simulink model "s_c_nbe_m32k"  (R2018a)
settings: Solver=VariableStepDiscrete  StartTime=0.0  StopTime=1000  RelTol=1e-3
undefined symbols (not defined in the file): fft_stages, n_taps, output_bits, pfb_coeff_gen_calc, xengbits
libraries: xbsIndex_r4 x23714, casper_library_misc x17, xps_library x4, casper_library_scopes x4, xbsReplacements_r4 x4
(part 85 of 171)

== system s_c_nbe_m32k/nb_pfb/pfb_fir_generic1/pfb_fir_taps ==
  sync : Inport
  din : Inport  Port=2
  coeffs : Inport  Port=3
  en : Inport  Port=4
  arnold : Terminator
  bram_din : xbsIndex_r4/Concat  num_inputs=2  dbl_ovrd=off  block_type=concat
  bus_adder_tree : Subsystem  mask(bus_adder_tree){n_busses=4, n_bits=[36 36], num_float_vec=1, bin_pts=34, dtypes=1, misc=off, floating_point=off, float_type=single, frac_width=24, exp_width=8, add_latency=7, first_stage_hdl=on, adder_imp=Behavioral}
      mask prompts: n_busses "number of busses"; n_bits "bus component bit widths"; num_float_vec "number floating point vectors in bus"; bin_pts "bus component binary points"; dtypes "bus component data types"; misc "misc support"; floating_point "floating point"; float_type "float type"; frac_width "fraction width"; exp_width "exponent width"; add_latency "adder latency"; first_stage_hdl "implement first stage in of adders in behavioral HDL?"; adder_imp "adder implementation"
      mask help: Add components of multiple identical busses
      mask init:
      | bus_adder_tree_init(gcb, ...
      |     'n_busses', n_busses, ...
      |     'n_bits', n_bits, ...
      |     'bin_pts', bin_pts, ...
      |     'dtypes', dtypes, ...
      |     'add_latency', add_latency, ...
      |     'floating_point', floating_point, ...
      |     'float_type', float_type, ...
      |     'exp_width', exp_width, ...
      |     'frac_width', frac_width, ...   
      |     'num_float_vec', num_float_vec, ...
      |     'first_stage_hdl', first_stage_hdl, ...
      |     'adder_imp', adder_imp, ...
      |     'misc', misc);
      mask Callback floating_point:
      | onoff = get_param(gcb, 'floating_point');
      | if strcmp(onoff,'on')
      |     enable_fixpt = 'off'
      |     set_param_state(gcb, 'float_type', 'on')
      |     set_param_state(gcb, 'num_float_vec', 'on')
      | 
      |     f_type = get_param(gcb, 'float_type')
      |     if strcmp(f_type,'custom')
      |         set_param_state(gcb, 'exp_width', 'on')
      |         set_param_state(gcb, 'frac_width', 'on')
      |     else
      |         set_param_state(gcb, 'exp_width', 'off')
      |         set_param_state(gcb, 'frac_width', 'off')
      |     end
      | 
      | 
      | else
      |     enable_fixpt = 'on'
      |     set_param_state(gcb, 'float_type', 'off')
      |     set_param_state(gcb, 'exp_width', 'off')
      |     set_param_state(gcb, 'frac_width', 'off')
      |     set_param_state(gcb, 'num_float_vec', 'off')
      | end
      | 
      | set_param_state(gcb, 'n_bits', enable_fixpt)
      | set_param_state(gcb, 'bin_pts', enable_fixpt)
      | set_param_state(gcb, 'dtypes', enable_fixpt)
      mask TypeOptions float_type: single | custom
      mask Callback float_type:
      | f_type = get_param(gcb, 'float_type')
      | if strcmp(f_type,'custom')
      |     set_param_state(gcb, 'exp_width', 'on')
      |     set_param_state(gcb, 'frac_width', 'on')
      | else
      |     set_param_state(gcb, 'exp_width', 'off')
      |     set_param_state(gcb, 'frac_width', 'off')
      | end
      mask TypeOptions adder_imp: Behavioral | Fabric | DSP48
  bus_mult : Subsystem  mask(bus_mult){n_bits_a=[18 18 18 18 18 18 18 18], bin_pt_a=17, type_a=1, cmplx_a=off, n_bits_b=[18 18 18 18 18 18 18 18], bin_pt_b=17, type_b=1, cmplx_b=off, misc=off, floating_point=off, float_type=single, input_vec_a=1, input_vec_b=1, frac_width=24, exp_width=8, n_bits_out=n_bits_data+n_bits_coeff, bin_pt_out=n_bits_data-1+bin_pt_coeff, type_out=1, quantization=0, overflow=0, mult_latency=mult_latency, add_latency=0, conv_latency=0, max_fanout=1, fan_latency=0, multiplier_implementation=behavioral HDL, pipeline_cmult_en=off, pipeline_latency=0}
      mask prompts: n_bits_a "a input bit widths"; bin_pt_a "a input binary points"; type_a "a input type (Unsigned=0, Signed=1)"; cmplx_a "a input complex"; n_bits_b "b input bit widths"; bin_pt_b "b input binary points"; type_b "b input type (Unsigned=0, Signed=1)"; cmplx_b "b input complex"; misc "misc support"; floating_point "floating point"; float_type "float type"; input_vec_a "a input vector in bus"; input_vec_b "b input vector in bus"; frac_width "fraction width"; exp_width "exponent width"; n_bits_out "output bit widths"; bin_pt_out "output binary points"; type_out "output type (Unsigned=0, Signed=1)"; quantization "quantization strategy (Truncate=0, Round  (unbiased: +/- Inf)=1)"; overflow "overflow strategy (Wrap=0, Saturate=1, Flag as error=2)"; mult_latency "multiplier latency"; add_latency "adder latency"; conv_latency "convert latency"; max_fanout "limit fanout to ?"; fan_latency "fanout register latency"; multiplier_implementation "multiplier implementation"; pipeline_cmult_en "pipeline complex mult"; pipeline_latency "pipeline latency"
      mask help: Multiply components of two busses
      mask init: same as s_c_nbe_m32k/DDC/bus_mult
      mask Callback floating_point:
      | onoff = get_param(gcb, 'floating_point');
      | if strcmp(onoff,'on')
      |     enable_fixpt = 'off'
      |     set_param_state(gcb, 'float_type', 'on')
      | 
      |     set_param_state(gcb, 'input_vec_a', 'on')
      |     set_param_state(gcb, 'input_vec_b', 'on')
      | 
      |     f_type = get_param(gcb, 'float_type')
      |     if strcmp(f_type,'custom')
      |         set_param_state(gcb, 'exp_width', 'on')
      |         set_param_state(gcb, 'frac_width', 'on')
      |     else
      |         set_param_state(gcb, 'exp_width', 'off')
      |         set_param_state(gcb, 'frac_width', 'off')
      |     end
      | 
      | else
      |     enable_fixpt = 'on'
      |     set_param_state(gcb, 'float_type', 'off')
      |     set_param_state(gcb, 'exp_width', 'off')
      |     set_param_state(gcb, 'frac_width', 'off')
      |     set_param_state(gcb, 'input_vec_a', 'off')
      |     set_param_state(gcb, 'input_vec_b', 'off')
      | end
      | 
      | set_param_state(gcb, 'n_bits_a', enable_fixpt)
      | set_param_state(gcb, 'bin_pt_a', enable_fixpt)
      | set_param_state(gcb, 'type_a', enable_fixpt)
      | set_param_state(gcb, 'n_bits_b', enable_fixpt)
      | set_param_state(gcb, 'bin_pt_b', enable_fixpt)
      | set_param_state(gcb, 'type_b', enable_fixpt)
      | 
      | set_param_state(gcb, 'n_bits_out', enable_fixpt)
      | set_param_state(gcb, 'bin_pt_out', enable_fixpt)
      | set_param_state(gcb, 'type_out', enable_fixpt)
      | set_param_state(gcb, 'quantization', enable_fixpt)
      | set_param_state(gcb, 'overflow', enable_fixpt)
      mask TypeOptions float_type: single | custom
      mask Callback float_type:
      | f_type = get_param(gcb, 'float_type')
      | if strcmp(f_type,'custom')
      |     set_param_state(gcb, 'exp_width', 'on')
      |     set_param_state(gcb, 'frac_width', 'on')
      | else
      |     set_param_state(gcb, 'exp_width', 'off')
      |     set_param_state(gcb, 'frac_width', 'off')
      | end
      mask TypeOptions multiplier_implementation: behavioral HDL | standard core | embedded multiplier core
      mask Callback pipeline_cmult_en:
      | pipeline_en = get_param(gcb, 'pipeline_cmult_en');
      | if strcmp(pipeline_en,'on')
      | 
      |     set_param_state(gcb, 'pipeline_latency', 'on')
      | else
      |     set_param_state(gcb, 'pipeline_latency', 'off')
      | end
  counter : xbsIndex_r4/Counter  cnt_type=Free Running  cnt_to=Inf  operation=Up  start_count=0  cnt_by_val=1  arith_type=Unsigned  n_bits=15  bin_pt=0  load_pin=off  rst=on  en=on  explicit_period=on  period=1  use_behavioral_HDL=off  implementation=Fabric  dbl_ovrd=off  block_type=counter
  daddr : xbsIndex_r4/Delay  rst=off  infoeditControl=Selection of Reset will increase slice count due to use of real FFs and instead of SRLs  en=off  latency=11  reg_retiming=on  dbl_ovrd=off  block_type=delay
  dcoeffs : xbsIndex_r4/Delay  rst=off  infoeditControl=Selection of Reset will increase slice count due to use of real FFs and instead of SRLs  en=off  latency=11  reg_retiming=on  dbl_ovrd=off  block_type=delay
  ddin : xbsIndex_r4/Delay  rst=off  infoeditControl=Selection of Reset will increase slice count due to use of real FFs and instead of SRLs  en=off  latency=11  reg_retiming=off  dbl_ovrd=off  block_type=delay
  den0 : xbsIndex_r4/Delay  rst=off  infoeditControl=Selection of Reset will increase slice count due to use of real FFs and instead of SRLs  en=off  latency=11  reg_retiming=on  dbl_ovrd=off  block_type=delay
  den1 : xbsIndex_r4/Delay  rst=off  infoeditControl=Selection of Reset will increase slice count due to use of real FFs and instead of SRLs  en=off  latency=7  reg_retiming=on  dbl_ovrd=off  block_type=delay
  den2 : xbsIndex_r4/Delay  rst=off  infoeditControl=Selection of Reset will increase slice count due to use of real FFs and instead of SRLs  en=off  latency=14  reg_retiming=on  dbl_ovrd=off  block_type=delay
  dsync0 : xbsIndex_r4/Delay  rst=off  infoeditControl=Selection of Reset will increase slice count due to use of real FFs and instead of SRLs  en=off  latency=11  reg_retiming=on  dbl_ovrd=off  block_type=delay
  dsync1 : xbsIndex_r4/Delay  rst=off  infoeditControl=Selection of Reset will increase slice count due to use of real FFs and instead of SRLs  en=off  latency=7  reg_retiming=on  dbl_ovrd=off  block_type=delay
  dsync2 : xbsIndex_r4/Delay  rst=off  infoeditControl=Selection of Reset will increase slice count due to use of real FFs and instead of SRLs  en=off  latency=14  reg_retiming=on  dbl_ovrd=off  block_type=delay
  mult_din : xbsIndex_r4/Concat  num_inputs=2  dbl_ovrd=off  block_type=concat
  never : xbsIndex_r4/Constant  const=0  gui_display_data_type=Fixed-point  arith_type=Boolean  n_bits=16  bin_pt=14  preci_type=Single  exp_width=8  frac_width=24  explicit_period=on  period=1  equ=P=C  opselect=C  inp2=PCIN>>17  opr=+  inp1=P  carry=CIN  dbl_ovrd=off  block_type=constant
  sync_delay1 : Subsystem  mask(sync_delay_en){DelayLen=(2^(pfb_size-n_inputs))*(n_taps-1)}
      mask prompts: DelayLen "Delay Length:"
      mask help: Delay an infrequent boolean pulse by the specified number of enabled clocks.
      mask init:
      | BitWidth = max(2, ceil(log2(DelayLen+1)));
      | UseCounter = 1;
      | if DelayLen == 0,
      | 	UseCounter = 0;
      | end
      mask Help: eval('xlWeb(''http://casper.berkeley.edu/wiki/Sync_delay_en'')')
      mask Display:
      | fprintf('Z^-%d', DelayLen);
      | port_label('input',2,'en');
  tap_delays : Subsystem  mask(bus_dual_port_ram){n_bits=[18 18 18 18 18 18], bin_pts=[0 0 0 0 0 0], init_vector=repmat(zeros(32768, 1), 1, 6), max_fanout=1, mem_type=Block RAM, bram_optimization=Speed, async_a=off, async_b=off, b_to_a_ratio_bits=0, misc=off, bram_latency=7, fan_latency=4, addra_register=on, addra_implementation=core, dina_register=off, dina_implementation=behavioral, wea_register=off, wea_implementation=behavioral, ena_register=off, ena_implementation=behavioral, addrb_register=on, addrb_implementation=core, dinb_register=on, dinb_implementation=core, web_register=on, web_implementation=core, enb_register=off, enb_implementation=behavioral}
      mask prompts: n_bits "data word bit widths"; bin_pts "data word binary points"; init_vector "initial value vector"; max_fanout "limit fanout to ?"; mem_type "memory type"; bram_optimization "memory optimization"; async_a "a asynchronous"; async_b "b asynchronous"; b_to_a_ratio_bits "b_to_a ratio bits"; misc "misc support"; bram_latency "bram latency"; fan_latency "input register latency"; addra_register "addra input register"; addra_implementation "addra register implementation"; dina_register "dina input register"; dina_implementation "dina register implementation"; wea_register "wea input register"; wea_implementation "wea register implementation"; ena_register "ena input register"; ena_implementation "ena register implementation"; addrb_register "addrb input register"; addrb_implementation "addrb register implementation"; dinb_register "dinb input register"; dinb_implementation "dinb register implementation"; web_register "web input register"; web_implementation "web register implementation"; enb_register "enb input register"; enb_implementation "enb register implementation"
      mask help: RAM for a bus allowing fanout control
      mask init: same as s_c_nbe_m32k/nb_pfb/pfb_fir_generic1/pfb_fir_coeff_gen/rom
      mask TypeOptions mem_type: Distributed memory | Block RAM
      mask TypeOptions bram_optimization: Area | Speed
      mask TypeOptions addra_implementation: core | behavioral
      mask TypeOptions dina_implementation: core | behavioral
      mask TypeOptions wea_implementation: core | behavioral
      mask TypeOptions ena_implementation: core | behavioral
      mask TypeOptions addrb_implementation: core | behavioral
      mask TypeOptions dinb_implementation: core | behavioral
      mask TypeOptions web_implementation: core | behavioral
      mask TypeOptions enb_implementation: core | behavioral
  tap_split : Subsystem  mask(bus_expand){mode=divisions of equal size, outputNum=4, outputWidth=72, outputBinaryPt=0, outputArithmeticType=0, show_format=off, outputToWorkspace=off, variablePrefix=out, outputToModelAsWell=on}
      mask prompts: outputNum "Number of outputs:"; outputWidth "Output width:"; outputBinaryPt "Output binary point position:"; outputArithmeticType "Output arithmetic type (ufix=0, fix=1, bool=2):"; show_format "Print format string?"; outputToWorkspace "Output to workspace?"; variablePrefix "Variable name prefix:"; outputToModelAsWell "Output to model as well?"
      mask help:
      | Expands a 'bus' made using a bus_create or Xilinx
      | concat block.
      | The input will be divided into the specified number
      | of outputs with the specified arithmetic types.
      | Divisions are made from most significant bit.
      mask init: same as s_c_nbe_m32k/bus_expand1
      settings: AttributesFormatString=4 outputs
      mask TypeOptions mode: divisions of equal size | divisions of arbitrary size
      mask Callback mode: bus_expand_callback();
      mask Callback outputWidth: bus_expand_callback();
      mask Callback outputToWorkspace: bus_expand_callback();
  youngest : xbsIndex_r4/Slice  nbits=(2*n_bits_data)*(n_taps-2)*(2^n_inputs)*n_streams  boolean_output=off  mode=Upper Bit Location + Width  bit1=0  base1=MSB of Input  bit0=0  base0=LSB of Input  dbl_ovrd=off  block_type=slice
  sync_out : Outport
  dout : Outport  Port=2
  dvalid : Outport  Port=3
  wires:
  dsync0/1 -> dsync1/1
  dsync1/1 -> dsync2/1
  dsync2/1 -> sync_out/1
  din/1 -> ddin/1
  coeffs/1 -> dcoeffs/1
  en/1 -> sync_delay1/2(en), den0/1, counter/2
  den0/1 -> den1/1, tap_delays/6(web)
  den1/1 -> den2/1
  sync/1 -> sync_delay1/1(In), counter/1
  sync_delay1/1(Out) -> dsync0/1
  ddin/1 -> bram_din/1, mult_din/1
  youngest/1 -> bram_din/2
  counter/1 -> daddr/1, tap_delays/1(addra)
  bram_din/1 -> tap_delays/2(dina), tap_delays/5(dinb)
  never/1 -> tap_delays/3(wea)
  daddr/1 -> tap_delays/4(addrb)
  tap_delays/2(B) -> arnold/1
  tap_delays/1(A) -> mult_din/2, youngest/1
  mult_din/1 -> bus_mult/1(a)
  dcoeffs/1 -> bus_mult/2(b)
  bus_mult/1(a*b) -> tap_split/1(bus_in)
  tap_split/1(msb_out4) -> bus_adder_tree/1(d0)
  tap_split/2(out3) -> bus_adder_tree/2(d1)
  tap_split/3(out2) -> bus_adder_tree/3(d2)
  tap_split/4(lsb_out1) -> bus_adder_tree/4(d3)
  bus_adder_tree/1(out) -> dout/1
  den2/1 -> dvalid/1

== system s_c_nbe_m32k/nb_pfb/pfb_fir_generic2/bus_convert ==
  din : Inport
  bussify : Subsystem  mask(bus_create){inputNum=2}
      mask prompts: inputNum "Number of inputs:"
      mask init:
      | bus_create_init(gcb,...
      |     'inputNum', inputNum);
  conv1 : Subsystem  mask(convert){bin_pt_in=35, n_bits_out=18, bin_pt_out=17, quantization=Round  (unbiased: +/- Inf), overflow=Wrap, csp_latency=4}
      mask prompts: bin_pt_in "Binary Point In"; n_bits_out "Bit Width Out"; bin_pt_out "Binary Point Out"; csp_latency "Latency"
      mask help:
      | Convert input value to the specified bit width and precision.
      |
      | Does not support upscaling number of fractional bits (eg 8_5 to 8_4 is ok, but not 8_4 to 8_5).
      mask init: same as s_c_nbe_m32k/cwg_cos/bus_convert/conv1
      settings: AttributesFormatString=|
      | N_35 ==> 18_17
      | round inf, wrap
      | latency = 4
      mask Help:
      | <pre>
      | Description::
      | 
      | Outputs converted version of the input.
      | 
      | Mask Parameters::
      | 
      | Binary Point In (bin_pt_in): Specifies the binary point location in the input.
      | 
      | Bit Width Out (n_bits_out): Specifies the width of the output.
      | 
      | Binary Point Out (bin_pt_out): Specifies the binary point location in the output.
      | 
      | Quantization (quantization): Specifies quantization handling.
      | 
      | Overflow (overflow): Specifies overflow handling.
      | 
      | Latency (latency): Specifies the latency of the underlying adder block, which is the overall
      | latency of this block as well.
      | </pre>
      mask TypeOptions quantization: Truncate | Round  (unbiased: +/- Inf) | Round  (unbiased: Even Values) | Round  (unbiased: Zero) | Round  (unbiased: Odd Values) | Round  (biased: Up) | Round  (biased: Down)
      mask TypeOptions overflow: Wrap | Saturate | Error
  conv2 : Subsystem  mask(convert){bin_pt_in=35, n_bits_out=18, bin_pt_out=17, quantization=Round  (unbiased: +/- Inf), overflow=Wrap, csp_latency=4}
      mask prompts: bin_pt_in "Binary Point In"; n_bits_out "Bit Width Out"; bin_pt_out "Binary Point Out"; csp_latency "Latency"
      mask help:
      | Convert input value to the specified bit width and precision.
      |
      | Does not support upscaling number of fractional bits (eg 8_5 to 8_4 is ok, but not 8_4 to 8_5).
      mask init: same as s_c_nbe_m32k/cwg_cos/bus_convert/conv1
      settings: AttributesFormatString=|
      | N_35 ==> 18_17
      | round inf, wrap
      | latency = 4
      mask Help:
      | <pre>
      | Description::
      | 
      | Outputs converted version of the input.
      | 
      | Mask Parameters::
      | 
      | Binary Point In (bin_pt_in): Specifies the binary point location in the input.
      | 
      | Bit Width Out (n_bits_out): Specifies the width of the output.
      | 
      | Binary Point Out (bin_pt_out): Specifies the binary point location in the output.
      | 
      | Quantization (quantization): Specifies quantization handling.
      | 
      | Overflow (overflow): Specifies overflow handling.
      | 
      | Latency (latency): Specifies the latency of the underlying adder block, which is the overall
      | latency of this block as well.
      | </pre>
      mask TypeOptions quantization: Truncate | Round  (unbiased: +/- Inf) | Round  (unbiased: Even Values) | Round  (unbiased: Zero) | Round  (unbiased: Odd Values) | Round  (biased: Up) | Round  (biased: Down)
      mask TypeOptions overflow: Wrap | Saturate | Error
  debus : Subsystem  mask(bus_expand){mode=divisions of arbitrary size, outputNum=1, outputWidth=[38 38], outputBinaryPt=[35 35], outputArithmeticType=[1 1], show_format=on, outputToWorkspace=off, variablePrefix=, outputToModelAsWell=on}
      mask prompts: outputNum "Number of outputs:"; outputWidth "Output width [msb ... lsb]:"; outputBinaryPt "Output binary point position [msb ... lsb]:"; outputArithmeticType "Output arithmetic type (ufix=0, fix=1, bool=2) [msb ... lsb]:"; show_format "Print format string?"; outputToWorkspace "Output to workspace?"; variablePrefix "Variable name prefix:"; outputToModelAsWell "Output to model as well?"
      mask help:
      | Expands a 'bus' made using a bus_create or Xilinx
      | concat block.
      | The input will be divided into the specified number
      | of outputs with the specified arithmetic types.
      | Divisions are made from most significant bit.
      mask init: same as s_c_nbe_m32k/bus_expand1
      settings: AttributesFormatString=2 outputs: f38.35,f38.35,
      mask TypeOptions mode: divisions of equal size | divisions of arbitrary size
      mask Callback mode: bus_expand_callback();
      mask Callback outputWidth: bus_expand_callback();
      mask Callback outputToWorkspace: bus_expand_callback();
  dout : Outport
  wires:
  bussify/1(bus_out) -> dout/1
  conv2/1(out) -> bussify/2(in2)
  conv1/1(out) -> bussify/1(in1)
  debus/2(lsb_out1) -> conv2/1(in)
  debus/1(msb_out2) -> conv1/1(in)
  din/1 -> debus/1(bus_in)

== system s_c_nbe_m32k/nb_pfb/pfb_fir_generic2/bus_create ==
  in1 : Inport
  reinterpret1 : xbsIndex_r4/Reinterpret  force_arith_type=on  arith_type=Unsigned  force_bin_pt=on  bin_pt=0  block_type=reinterpret
      settings: infoedit="Changes signal type without altering the binary representation.   You can changed the signal between signed and unsigned, and relocate the binary point.<br><br>Hardware notes: In hardware this block costs nothing.<br><br>Example:  Suppose the input is 6 bits wide, signed, with 2 fractional bits, and the output is forced to unsigned with 0 fractional bits.  Then an input of -2.0 (1110.00 in binary 2's complement) becomes an output of 56 (111000 in binary)."
  bus_out : Outport
  wires:
  reinterpret1/1 -> bus_out/1
  in1/1 -> reinterpret1/1

== system s_c_nbe_m32k/nb_pfb/pfb_fir_generic2/bus_expand ==
  bus_in : Inport
  reinterpret1 : xbsIndex_r4/Reinterpret  force_arith_type=on  arith_type=Unsigned  force_bin_pt=on  bin_pt=0  block_type=reinterpret
  slice1 : xbsIndex_r4/Slice  nbits=36  boolean_output=off  mode=Upper Bit Location + Width  bit1=0  base1=MSB of Input  bit0=0  base0=LSB of Input  dbl_ovrd=off  block_type=slice
  msb_lsb_out1 : Outport
  wires:
  reinterpret1/1 -> msb_lsb_out1/1
  slice1/1 -> reinterpret1/1
  bus_in/1 -> slice1/1

== system s_c_nbe_m32k/nb_pfb/pfb_fir_generic2/bus_scale ==
  din : Inport
  bussify : Subsystem  mask(bus_create){inputNum=2}
      mask prompts: inputNum "Number of inputs:"
      mask init:
      | bus_create_init(gcb,...
      |     'inputNum', inputNum);
  debus : Subsystem  mask(bus_expand){mode=divisions of arbitrary size, outputNum=1, outputWidth=[38 38], outputBinaryPt=[34 34], outputArithmeticType=[1 1], show_format=on, outputToWorkspace=off, variablePrefix=, outputToModelAsWell=on}
      mask prompts: outputNum "Number of outputs:"; outputWidth "Output width [msb ... lsb]:"; outputBinaryPt "Output binary point position [msb ... lsb]:"; outputArithmeticType "Output arithmetic type (ufix=0, fix=1, bool=2) [msb ... lsb]:"; show_format "Print format string?"; outputToWorkspace "Output to workspace?"; variablePrefix "Variable name prefix:"; outputToModelAsWell "Output to model as well?"
      mask help:
      | Expands a 'bus' made using a bus_create or Xilinx
      | concat block.
      | The input will be divided into the specified number
      | of outputs with the specified arithmetic types.
      | Divisions are made from most significant bit.
      mask init: same as s_c_nbe_m32k/bus_expand1
      settings: AttributesFormatString=2 outputs: f38.34,f38.34,
      mask TypeOptions mode: divisions of equal size | divisions of arbitrary size
      mask Callback mode: bus_expand_callback();
      mask Callback outputWidth: bus_expand_callback();
      mask Callback outputToWorkspace: bus_expand_callback();
  scale1 : xbsIndex_r4/Scale  scale_factor=-1  dbl_ovrd=off  block_type=scale
  scale2 : xbsIndex_r4/Scale  scale_factor=-1  dbl_ovrd=off  block_type=scale
  dout : Outport
  wires:
  bussify/1(bus_out) -> dout/1
  scale2/1 -> bussify/2(in2)
  scale1/1 -> bussify/1(in1)
  debus/2(lsb_out1) -> scale2/1
  debus/1(msb_out2) -> scale1/1
  din/1 -> debus/1(bus_in)

== system s_c_nbe_m32k/nb_pfb/pfb_fir_generic2/coeff_munge ==
  din : Inport
  join : Subsystem  mask(bus_create){inputNum=8}
      mask prompts: inputNum "Number of inputs:"
      mask init:
      | bus_create_init(gcb,...
      |     'inputNum', inputNum);
  reinterpret : xbsIndex_r4/Reinterpret  force_arith_type=on  arith_type=Unsigned  force_bin_pt=on  bin_pt=0  block_type=reinterpret
  reinterpret_out : xbsIndex_r4/Reinterpret  force_arith_type=on  arith_type=Unsigned  force_bin_pt=on  bin_pt=0  block_type=reinterpret
  split : Subsystem  mask(bus_expand){mode=divisions of arbitrary size, outputNum=1, outputWidth=[18 18 18 18], outputBinaryPt=[0 0 0 0], outputArithmeticType=[0 0 0 0], show_format=off, outputToWorkspace=off, variablePrefix=out, outputToModelAsWell=on}
      mask prompts: outputNum "Number of outputs:"; outputWidth "Output width [msb ... lsb]:"; outputBinaryPt "Output binary point position [msb ... lsb]:"; outputArithmeticType "Output arithmetic type (ufix=0, fix=1, bool=2) [msb ... lsb]:"; show_format "Print format string?"; outputToWorkspace "Output to workspace?"; variablePrefix "Variable name prefix:"; outputToModelAsWell "Output to model as well?"
      mask help:
      | Expands a 'bus' made using a bus_create or Xilinx
      | concat block.
      | The input will be divided into the specified number
      | of outputs with the specified arithmetic types.
      | Divisions are made from most significant bit.
      mask init: same as s_c_nbe_m32k/bus_expand1
      settings: AttributesFormatString=4 outputs
      mask TypeOptions mode: divisions of equal size | divisions of arbitrary size
      mask Callback mode: bus_expand_callback();
      mask Callback outputWidth: bus_expand_callback();
      mask Callback outputToWorkspace: bus_expand_callback();
  dout : Outport
  wires:
  split/1(msb_out4) -> join/8(in8), join/7(in7)
  split/2(out3) -> join/6(in6), join/5(in5)
  split/3(out2) -> join/4(in4), join/3(in3)
  split/4(lsb_out1) -> join/2(in2), join/1(in1)
  join/1(bus_out) -> reinterpret_out/1
  reinterpret/1 -> split/1(bus_in)
  din/1 -> reinterpret/1
  reinterpret_out/1 -> dout/1

== system s_c_nbe_m32k/nb_pfb/pfb_fir_generic2/pfb_fir_coeff_gen ==
  sync : Inport
  din : Inport  Port=2
  en : Inport  Port=3
  a_expand : Subsystem  AncestorBlock=casper_library_flow_control/bus_expand  mask(bus_expand){mode=divisions of equal size, outputNum=2, outputWidth=18, outputBinaryPt=0, outputArithmeticType=0, show_format=off, outputToWorkspace=off, variablePrefix=out, outputToModelAsWell=on}
      mask prompts: outputNum "Number of outputs:"; outputWidth "Output width:"; outputBinaryPt "Output binary point position:"; outputArithmeticType "Output arithmetic type (ufix=0, fix=1, bool=2):"; show_format "Print format string?"; outputToWorkspace "Output to workspace?"; variablePrefix "Variable name prefix:"; outputToModelAsWell "Output to model as well?"
      mask help:
      | Expands a 'bus' made using a bus_create or Xilinx
      | concat block.
      | The input will be divided into the specified number
      | of outputs with the specified arithmetic types.
      | Divisions are made from most significant bit.
      mask init: same as s_c_nbe_m32k/bus_expand1
      settings: AttributesFormatString=2 outputs
      mask TypeOptions mode: divisions of equal size | divisions of arbitrary size
      mask Callback mode: bus_expand_callback();
      mask Callback outputWidth: bus_expand_callback();
      mask Callback outputToWorkspace: bus_expand_callback();
  b_expand : Subsystem  AncestorBlock=casper_library_flow_control/bus_expand  mask(bus_expand){mode=divisions of equal size, outputNum=2, outputWidth=18, outputBinaryPt=0, outputArithmeticType=0, show_format=off, outputToWorkspace=off, variablePrefix=out, outputToModelAsWell=on}
      mask prompts: outputNum "Number of outputs:"; outputWidth "Output width:"; outputBinaryPt "Output binary point position:"; outputArithmeticType "Output arithmetic type (ufix=0, fix=1, bool=2):"; show_format "Print format string?"; outputToWorkspace "Output to workspace?"; variablePrefix "Variable name prefix:"; outputToModelAsWell "Output to model as well?"
      mask help:
      | Expands a 'bus' made using a bus_create or Xilinx
      | concat block.
      | The input will be divided into the specified number
      | of outputs with the specified arithmetic types.
      | Divisions are made from most significant bit.
      mask init: same as s_c_nbe_m32k/bus_expand1
      settings: AttributesFormatString=2 outputs
      mask TypeOptions mode: divisions of equal size | divisions of arbitrary size
      mask Callback mode: bus_expand_callback();
      mask Callback outputWidth: bus_expand_callback();
      mask Callback outputToWorkspace: bus_expand_callback();
  concat : xbsIndex_r4/Concat  num_inputs=4  dbl_ovrd=off  block_type=concat
  const0 : xbsIndex_r4/Constant  const=1  gui_display_data_type=Fixed-point  arith_type=Signed (2's comp)  n_bits=18  bin_pt=17  preci_type=Single  exp_width=8  frac_width=24  explicit_period=on  period=1  equ=P=C  opselect=C  inp2=PCIN>>17  opr=+  inp1=P  carry=CIN  dbl_ovrd=off  block_type=constant
  const1 : xbsIndex_r4/Constant  const=1.949e-17  gui_display_data_type=Fixed-point  arith_type=Signed (2's comp)  n_bits=18  bin_pt=17  preci_type=Single  exp_width=8  frac_width=24  explicit_period=on  period=1  equ=P=C  opselect=C  inp2=PCIN>>17  opr=+  inp1=P  carry=CIN  dbl_ovrd=off  block_type=constant
  counter : xbsIndex_r4/Counter  cnt_type=Free Running  cnt_to=Inf  operation=Up  start_count=0  cnt_by_val=1  arith_type=Unsigned  n_bits=15  bin_pt=0  load_pin=off  rst=on  en=on  explicit_period=on  period=1  use_behavioral_HDL=off  implementation=Fabric  dbl_ovrd=off  block_type=counter
  d0 : xbsIndex_r4/Delay  rst=off  infoeditControl=Selection of Reset will increase slice count due to use of real FFs and instead of SRLs  en=off  latency=1  reg_retiming=on  dbl_ovrd=off  block_type=delay
  d1 : xbsIndex_r4/Delay  rst=off  infoeditControl=Selection of Reset will increase slice count due to use of real FFs and instead of SRLs  en=off  latency=1  reg_retiming=on  dbl_ovrd=off  block_type=delay
  d2 : xbsIndex_r4/Delay  rst=off  infoeditControl=Selection of Reset will increase slice count due to use of real FFs and instead of SRLs  en=on  latency=1  reg_retiming=on  dbl_ovrd=off  block_type=delay
  d3 : xbsIndex_r4/Delay  rst=off  infoeditControl=Selection of Reset will increase slice count due to use of real FFs and instead of SRLs  en=on  latency=1  reg_retiming=on  dbl_ovrd=off  block_type=delay
  den0 : xbsIndex_r4/Delay  rst=off  infoeditControl=Selection of Reset will increase slice count due to use of real FFs and instead of SRLs  en=off  latency=11  reg_retiming=on  dbl_ovrd=off  block_type=delay
  den1 : xbsIndex_r4/Delay  rst=off  infoeditControl=Selection of Reset will increase slice count due to use of real FFs and instead of SRLs  en=off  latency=1  reg_retiming=on  dbl_ovrd=off  block_type=delay
  dfirst : xbsIndex_r4/Delay  rst=off  infoeditControl=Selection of Reset will increase slice count due to use of real FFs and instead of SRLs  en=off  latency=7  reg_retiming=on  dbl_ovrd=off  block_type=delay
  din_delay : xbsIndex_r4/Delay  rst=off  infoeditControl=Selection of Reset will increase slice count due to use of real FFs and instead of SRLs  en=off  latency=12  reg_retiming=on  dbl_ovrd=off  block_type=delay
  first : xbsIndex_r4/Relational  mode=a=b  op_type=Bool  en=off  latency=4  dbl_ovrd=off  block_type=relational
  inverter : xbsIndex_r4/Inverter  en=off  latency=0  dbl_ovrd=off  block_type=inv
  munge : Subsystem  AncestorBlock=casper_library_flow_control/munge  mask(munge){divisions=2, div_size=[18 18], order=[1 0], arith_type_out=Unsigned, bin_pt_out=0}
      mask prompts: divisions "Number of divisions"; div_size "Division size (bits)"; order "Division packing order"; arith_type_out "Output arithmetic type"; bin_pt_out "Output binary point"
      mask help: Splits an input bus into the specified number of divisions and then recombines them in the order specified (most significant division = 0,least = number divisions-1)
      mask init:
      | munge_init(gcb, ...
      |     'divisions', divisions, ...
      |     'div_size', div_size, ...
      |     'order', order, ...
      |     'arith_type_out', arith_type_out, ...
      |     'bin_pt_out', bin_pt_out);
      settings: AttributesFormatString=|
      | split:[18 18]
      | join:[1 0]
      | Unsigned [36,0]
      mask TypeOptions arith_type_out: Unsigned | Signed  (2's comp) | Floating-point
  mux0 : xbsIndex_r4/Mux  inputs=2  en=off  latency=1  precision=Full  arith_type=Unsigned  n_bits=16  bin_pt=14  quantization=Truncate  overflow=Wrap  dbl_ovrd=off  block_type=mux
  mux1 : xbsIndex_r4/Mux  inputs=2  en=off  latency=1  precision=Full  arith_type=Unsigned  n_bits=16  bin_pt=14  quantization=Truncate  overflow=Wrap  dbl_ovrd=off  block_type=mux
  reinterpret0 : xbsIndex_r4/Reinterpret  force_arith_type=on  arith_type=Unsigned  force_bin_pt=on  bin_pt=0  block_type=reinterpret
  reinterpret1 : xbsIndex_r4/Reinterpret  force_arith_type=on  arith_type=Unsigned  force_bin_pt=on  bin_pt=0  block_type=reinterpret
  rom : Subsystem  AncestorBlock=casper_library_bus/bus_dual_port_ram  mask(bus_dual_port_ram){n_bits=[18 18], bin_pts=[17 17], init_vector=[pfb_coeff_gen_calc(15, 4, 'hann', 0, 0, 1, 1, false)', pfb_coeff_gen_calc(15, 4, 'hann', 0, 0, 1, 2, false)'], max_fanout=1, mem_type=Block RAM, bram_optimization=Speed, async_a=off, async_b=off, b_to_a_ratio_bits=0, misc=off, bram_latency=7, fan_latency=4, addra_register=on, addra_implementation=core, dina_register=off, dina_implementation=behavioral, wea_register=off, wea_implementation=behavioral, ena_register=off, ena_implementation=core, addrb_register=on, addrb_implementation=core, dinb_register=off, dinb_implementation=behavioral, web_register=off, web_implementation=behavioral, enb_register=off, enb_implementation=core}
      mask prompts: n_bits "data word bit widths"; bin_pts "data word binary points"; init_vector "initial value vector"; max_fanout "limit fanout to ?"; mem_type "memory type"; bram_optimization "memory optimization"; async_a "a asynchronous"; async_b "b asynchronous"; b_to_a_ratio_bits "b_to_a ratio bits"; misc "misc support"; bram_latency "bram latency"; fan_latency "input register latency"; addra_register "addra input register"; addra_implementation "addra register implementation"; dina_register "dina input register"; dina_implementation "dina register implementation"; wea_register "wea input register"; wea_implementation "wea register implementation"; ena_register "ena input register"; ena_implementation "ena register implementation"; addrb_register "addrb input register"; addrb_implementation "addrb register implementation"; dinb_register "dinb input register"; dinb_implementation "dinb register implementation"; web_register "web input register"; web_implementation "web register implementation"; enb_register "enb input register"; enb_implementation "enb register implementation"
      mask help: RAM for a bus allowing fanout control
      mask init: same as s_c_nbe_m32k/nb_pfb/pfb_fir_generic1/pfb_fir_coeff_gen/rom
      mask TypeOptions mem_type: Distributed memory | Block RAM
      mask TypeOptions bram_optimization: Area | Speed
      mask TypeOptions addra_implementation: core | behavioral
      mask TypeOptions dina_implementation: core | behavioral
      mask TypeOptions wea_implementation: core | behavioral
      mask TypeOptions ena_implementation: core | behavioral
      mask TypeOptions addrb_implementation: core | behavioral
      mask TypeOptions dinb_implementation: core | behavioral
      mask TypeOptions web_implementation: core | behavioral
      mask TypeOptions enb_implementation: core | behavioral
  rom_din : xbsIndex_r4/Constant  const=0  gui_display_data_type=Fixed-point  arith_type=Unsigned  n_bits=36  bin_pt=0  preci_type=Single  exp_width=8  frac_width=24  explicit_period=on  period=1  equ=P=C  opselect=C  inp2=PCIN>>17  opr=+  inp1=P  carry=CIN  dbl_ovrd=off  block_type=constant
  rom_we : xbsIndex_r4/Constant  const=0  gui_display_data_type=Fixed-point  arith_type=Boolean  n_bits=16  bin_pt=14  preci_type=Single  exp_width=8  frac_width=24  explicit_period=on  period=1  equ=P=C  opselect=C  inp2=PCIN>>17  opr=+  inp1=P  carry=CIN  dbl_ovrd=off  block_type=constant
  sync_delay : xbsIndex_r4/Delay  rst=off  infoeditControl=Selection of Reset will increase slice count due to use of real FFs and instead of SRLs  en=off  latency=12  reg_retiming=on  dbl_ovrd=off  block_type=delay
  zero : xbsIndex_r4/Constant  const=0  gui_display_data_type=Fixed-point  arith_type=Unsigned  n_bits=15  bin_pt=0  preci_type=Single  exp_width=8  frac_width=24  explicit_period=on  period=1  equ=P=C  opselect=C  inp2=PCIN>>17  opr=+  inp1=P  carry=CIN  dbl_ovrd=off  block_type=constant
  sync_out : Outport
  dout : Outport  Port=2
  coeffs : Outport  Port=3
  dvalid : Outport  Port=4
  wires:
  sync/1 -> sync_delay/1, counter/1
  sync_delay/1 -> sync_out/1
  din/1 -> din_delay/1
  din_delay/1 -> dout/1
  counter/1 -> inverter/1, rom/1(addra), first/2
  inverter/1 -> rom/4(addrb)
  rom_din/1 -> rom/2(dina), rom/5(dinb)
  rom_we/1 -> rom/3(wea), rom/6(web)
  zero/1 -> first/1
  first/1 -> dfirst/1
  rom/2(B) -> munge/1(din)
  rom/1(A) -> a_expand/1(bus_in)
  munge/1(dout) -> b_expand/1(bus_in)
  concat/1 -> coeffs/1
  a_expand/1(msb_out2) -> d0/1
  d0/1 -> concat/1
  a_expand/2(lsb_out1) -> d1/1
  d1/1 -> concat/2
  b_expand/1(msb_out2) -> d2/1
  const0/1 -> reinterpret0/1
  reinterpret0/1 -> mux0/3
  dfirst/1 -> mux0/1, mux1/1
  d2/1 -> mux0/2
  mux0/1 -> concat/3
  b_expand/2(lsb_out1) -> d3/1
  const1/1 -> reinterpret1/1
  reinterpret1/1 -> mux1/3
  d3/1 -> mux1/2
  mux1/1 -> concat/4
  en/1 -> counter/2, den0/1
  den0/1 -> d2/2, d3/2, den1/1
  den1/1 -> dvalid/1
